simulink model "PumpDriverTestHarness"  (R2025b)
settings: Solver=VariableStepAuto  StartTime=0.0  StopTime=1200  RelTol=1e-3
PreLoadFcn:
  | PumpDriverTestHarnessParams;
undefined symbols (not defined in the file or in its folder): pumpDriver
libraries: fl_lib x13, nesl_utility x5, SimscapeFluids_lib x1
settings Model: Creator=jjha  LastModifiedBy=jjha
settings OptimizationCC: ReuseModelBlockBuffer=off
settings RTWCC: GPUComputeCapability=3.5
settings SimscapeCC: SimscapeLogType=all  SimscapeLogDataHistory=1000000.0

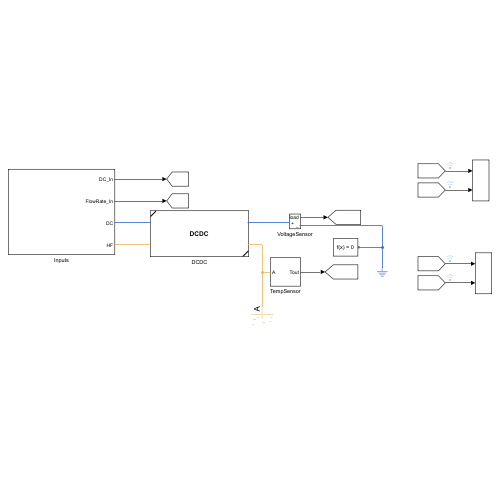
[thumbnail: Simulink's stored preview of the top-level diagram]
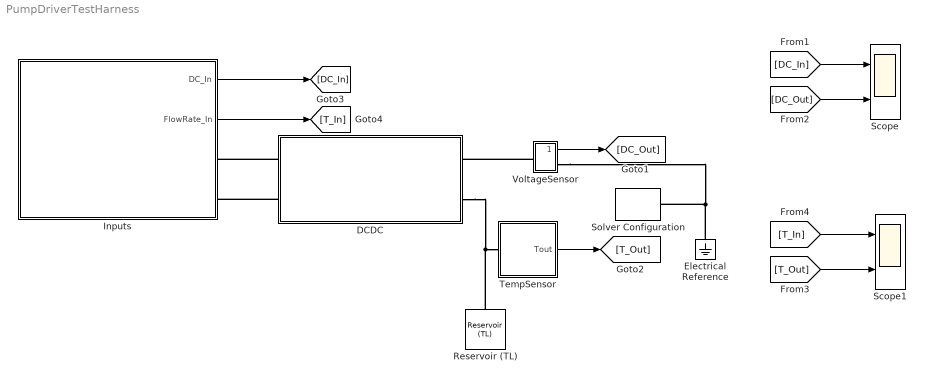
== system PumpDriverTestHarness ==
  DCDC : Subsystem  VariantControl=Driveline == 1  ReferencedSubsystem=PumpDriverTh
  Electrical Reference : fl_lib/Electrical/Electrical Elements/Electrical Reference
  Inputs : Subsystem
  Reservoir (TL) : fl_lib/Thermal Liquid/Elements/Reservoir (TL)  pressure_spec=foundation.enum.pressure_spec.atmospheric  reservoir_pressure=0.101325 MPa  reservoir_temperature=298 K  area=pi * pumpDriver.coolant_channel_D^2 / 4 m^2
  Scope : Scope  NumInputPorts=2
      settings: ActiveDisplayYMinimum=-150  ActiveDisplayYMaximum=1350
  Scope1 : Scope  NumInputPorts=2
      settings: ActiveDisplayYMinimum=298.11645  ActiveDisplayYMaximum=298.50196
  Solver Configuration : nesl_utility/Solver Configuration  PhysicalDomain=network_engine_domain  SubClassName=solver  LeftPortType=input  RightPortType=generic  Tones=[]  Harmonics=[]  SimulateNoise=off  Profile=off  UseLocalSampling=off  EnableSwitchedLinearOptims=on  FrequencyDomain=off  UseCCode=off  RelTol=0.001  AbsTol=0.001  MinStep=1e-09  ToWorkspace=off  RevertToSquareIcSolve=off  NumHomotopyIterations=100  PhasorMode=off  PhasorModeNumHarmonics=1  ConsistencySolver=NEWTON_XTOL_AFTER_FTOL  IndexReductionMethod=DerivativeReplacement  DoDC=off  ResidualTolerance=1e-09  ConsistencyTolSource=GLOBAL  ConsistencyAbsTol=0.001  ConsistencyRelTol=0.001  ConsistencyTolFactor=0.001  UseLocalSolver=off  LocalSolverChoice=NE_BACKWARD_EULER_ADVANCER  ResolveIndetEquations=on  FunctionEvalNumThread=1  LocalSolverSampleTime=0.001  DoFixedCost=off  MaxNonlinIter=3  MaxModeIter=2  ComputeImpulses=off  ImpulseIterations=2  LinearAlgebra=auto  LinearAlgebraNumThread=0  EquationFormulation=NE_TIME_EF  DelaysMemoryBudget=1024  AutomaticFiltering=on  FilteringTimeConstant=0.001  PartitionStorageMethod=AS_NEEDED  PartitionMemoryBudget=1024  PartitionMethod=ROBUST  MultibodyUseLocalSolver=off  MultibodyLocalSolverChoice=ODE1  MultibodyLocalSolverSampleTime=0.001
  TempSensor : Subsystem
  VoltageSensor : Subsystem
  wires:
  [DC_In] -> Scope/1
  [DC_Out] -> Scope/2
  VoltageSensor/1(load) -> [DC_Out]
  Inputs/1(DC_In) -> [DC_In]
  TempSensor/1(Tout) -> [T_Out]
  [T_Out] -> Scope1/2
  Inputs/2(FlowRate_In) -> [T_In]
  [T_In] -> Scope1/1
  connections:
  Electrical Reference/LConn1 -- VoltageSensor/RConn1 -- Solver Configuration/RConn1
  DCDC/LConn1 -- Inputs/RConn1
  DCDC/RConn2 -- Reservoir (TL)/LConn1 -- TempSensor/LConn1
  VoltageSensor/LConn1 -- DCDC/RConn1
  DCDC/LConn2 -- Inputs/RConn2

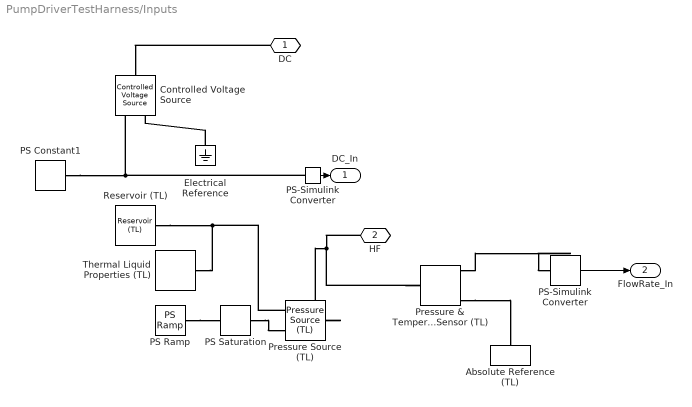
== system PumpDriverTestHarness/Inputs ==
  Absolute Reference (TL) : fl_lib/Thermal Liquid/Elements/Absolute Reference (TL)
  Controlled Voltage Source : fl_lib/Electrical/Electrical Sources/Controlled Voltage Source
  Electrical Reference : fl_lib/Electrical/Electrical Elements/Electrical Reference
  PS Constant1 : fl_lib/Physical Signals/Sources/PS Constant  constant=400
  PS Ramp : fl_lib/Physical Signals/Sources/PS Ramp  slope=16/1200 MPa/s  start_time=0 s  initial_output=0 MPa  ZeroCross=true
  PS Saturation : fl_lib/Physical Signals/Nonlinear Operators/PS Saturation  upper_limit=16 MPa  lower_limit=0 MPa  ZeroCross=true
  PS-Simulink Converter : nesl_utility/PS-Simulink Converter  PhysicalDomain=network_engine_domain  SubClassName=ps_output  LeftPortType=input  RightPortType=output  PseudoPeriodic=off  Frequencies=[]  VectorFormat=inherit  Unit=inherit  AffineConversion=off
  PS-Simulink Converter : nesl_utility/PS-Simulink Converter  PhysicalDomain=network_engine_domain  SubClassName=ps_output  LeftPortType=input  RightPortType=output  PseudoPeriodic=off  Frequencies=[]  VectorFormat=1-D array  Unit=1  AffineConversion=off
  Pressure & Temperature Sensor (TL) : fl_lib/Thermal Liquid/Sensors/Pressure & Temperature Sensor (TL)  reference=foundation.enum.MeasurementReference.difference  pressure=true  pressure_spec=foundation.enum.PressureMeasementSpec.Absolute  temperature=true
      settings: InternalSimscapePortConfiguration="{\"Bottom\":[{\"id\":\"T\",\"label\":\"T\",\"type\":\"output\"}],\"Left\":[{\"id\":\"A\",\"label\":\"A\",\"type\":\"foundation.thermal_liquid.thermal_liquid\"}],\"Right\":[{\"id\":\"B\",\"label\":\"B\",\"type\":\"foundation.thermal_liquid.thermal_liquid\"},{\"id\":\"P\",\"label\":\"P\",\"type\":\"output\"}],\"Top\":[]}"
  Pressure Source (TL) : fl_lib/Thermal Liquid/Sources/Pressure Source (TL)  source_type=foundation.enum.constant_controlled.controlled  pressure_differential=0 MPa  power_spec=foundation.enum.power_spec.isentropic  area=0.01 m^2
      settings: InternalSimscapePortConfiguration="{\"Bottom\":[],\"Left\":[{\"id\":\"A\",\"label\":\"A\",\"type\":\"foundation.thermal_liquid.thermal_liquid\"},{\"id\":\"P\",\"label\":\"P\",\"type\":\"input\"}],\"Right\":[{\"id\":\"B\",\"label\":\"B\",\"type\":\"foundation.thermal_liquid.thermal_liquid\"}],\"Top\":[]}"
  Reservoir (TL) : fl_lib/Thermal Liquid/Elements/Reservoir (TL)  pressure_spec=foundation.enum.pressure_spec.atmospheric  reservoir_pressure=0.101325 MPa  reservoir_temperature=vehicleThermal.coolant_T_init K  area=pi * pumpDriver.coolant_channel_D^2 / 4 m^2
  Thermal Liquid Properties (TL) : SimscapeFluids_lib/Thermal Liquid/Utilities/Thermal Liquid Properties (TL)  fluid_list=fluids.thermal_liquid.utilities.enum.thermal_liquid_fluid_list.water  concentration_param_EG=fluids.thermal_liquid.utilities.enum.thermal_liquid_concentration.volume_fraction  concentration_param_PG=fluids.thermal_liquid.utilities.enum.thermal_liquid_concentration.volume_fraction  c_mass_SW=3.5e-3  c_mass_EG=0.1  c_mass_PG=0.1  c_mass_GL=0.1  c_vol_EG=0.1  c_vol_PG=0.1  beta_const_EG=2.1791 GPa  beta_const_PG=2.1791 GPa  beta_const_GL=2.1791 GPa  p_min_EG=0.01 MPa  p_min_PG=0.01 MPa  p_min_GL=0.01 MPa  p_max_EG=50 MPa  p_max_PG=50 MPa  p_max_GL=50 MPa  p_atm=0.101325 MPa  properties_range_check=simscape.enum.assert.action.error
  DC : PMIOPort  Side=Right
  HF : PMIOPort  Port=2  Side=Right
  DC_In : Outport
  FlowRate_In : Outport  Port=2
  wires:
  PS-Simulink Converter/1 -> DC_In/1
  PS-Simulink Converter/1 -> FlowRate_In/1
  connections:
  DC/RConn1 -- Controlled Voltage Source/LConn1
  Electrical Reference/LConn1 -- Controlled Voltage Source/RConn2
  HF/RConn1 -- Pressure Source (TL)/RConn1 -- Pressure & Temperature Sensor (TL)/LConn1
  Reservoir (TL)/LConn1 -- Pressure Source (TL)/LConn1 -- Thermal Liquid Properties (TL)/RConn1
  PS Constant1/RConn1 -- PS-Simulink Converter/LConn1 -- Controlled Voltage Source/RConn1
  Pressure & Temperature Sensor (TL)/RConn1 -- Absolute Reference (TL)/LConn1
  Pressure & Temperature Sensor (TL)/RConn3 -- PS-Simulink Converter/LConn1
  PS Ramp/RConn1 -- PS Saturation/LConn1
  PS Saturation/RConn1 -- Pressure Source (TL)/LConn2

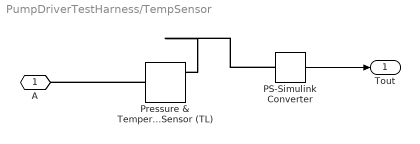
== system PumpDriverTestHarness/TempSensor ==
  PS-Simulink Converter : nesl_utility/PS-Simulink Converter  PhysicalDomain=network_engine_domain  SubClassName=ps_output  LeftPortType=input  RightPortType=output  PseudoPeriodic=off  Frequencies=[]  VectorFormat=1-D array  Unit=K  AffineConversion=off
  Pressure & Temperature Sensor (TL) : fl_lib/Thermal Liquid/Sensors/Pressure & Temperature Sensor (TL)  reference=foundation.enum.MeasurementReference.absolute  pressure=true  pressure_spec=foundation.enum.PressureMeasementSpec.Gauge  temperature=true
      settings: InternalSimscapePortConfiguration="{\"Bottom\":[{\"id\":\"T\",\"label\":\"T\",\"type\":\"output\"}],\"Left\":[{\"id\":\"A\",\"label\":\"A\",\"type\":\"foundation.thermal_liquid.thermal_liquid\"}],\"Right\":[{\"id\":\"Pg\",\"label\":\"Pg\",\"type\":\"output\"}],\"Top\":[]}"
  A : PMIOPort  Side=Left
  Tout : Outport
  wires:
  PS-Simulink Converter/1 -> Tout/1
  connections:
  Pressure & Temperature Sensor (TL)/LConn1 -- A/RConn1
  PS-Simulink Converter/LConn1 -- Pressure & Temperature Sensor (TL)/RConn2

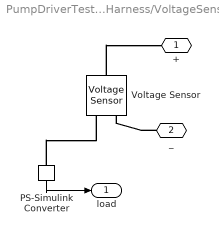
== system PumpDriverTestHarness/VoltageSensor ==
  PS-Simulink Converter : nesl_utility/PS-Simulink Converter  PhysicalDomain=network_engine_domain  SubClassName=ps_output  LeftPortType=input  RightPortType=output  PseudoPeriodic=off  Frequencies=[]  VectorFormat=inherit  Unit=inherit  AffineConversion=off
  Voltage Sensor : fl_lib/Electrical/Electrical Sensors/Voltage Sensor
  + : PMIOPort  Side=Left
  _ : PMIOPort  Port=2  Side=Right
  load : Outport
  wires:
  PS-Simulink Converter/1 -> load/1
  connections:
  PS-Simulink Converter/LConn1 -- Voltage Sensor/RConn1
  _/RConn1 -- Voltage Sensor/RConn2
  Voltage Sensor/LConn1 -- +/RConn1
